simulink model "line_follower_ir"  (R2024b)
settings: Solver=FixedStepDiscrete  StartTime=0.0  StopTime=inf  FixedStep=0.001  RelTol=1e-3  EnableMultiTasking=on
libraries: arduinolib x2
settings Model: ExtModeTrigDuration=2  Creator=$V8IK00-KEIKKPI1645J  LastModifiedBy=$V8IK00-KEIKKPI1645J
settings SolverCC: AutoInsertRateTranBlk=on
settings OptimizationCC: EnhancedBackFolding=on  PassReuseOutputArgsAs=Individual arguments  ZeroExternalMemoryAtStartup=off  ZeroInternalMemoryAtStartup=off  MaxStackSize=64  OptimizeBlockOrder=speed  DifferentSizesBufferReuse=on  OptimizationCustomize=off  EfficientTunableParamExpr=on
settings DebuggingCC: ParameterTunabilityLossMsg=error
settings HardwareCC: ProdBitPerInt=16  ProdBitPerPointer=16  ProdBitPerSizeT=16  ProdBitPerPtrDiffT=16  ProdLargestAtomicFloat=None  ProdWordSize=8  ProdHWDeviceType=Atmel->AVR
settings SFSimCC: MATLABDynamicMemAlloc=off
settings RTWCC: Description=Embedded Coder  SystemTargetFile=ert.tlc  HardwareBoard=Arduino Uno  TemplateMakefile=ert_default_tmf  Toolchain=Arduino AVR  BuildConfiguration=Faster Runs
settings CodeAppCC: ForceParamTrailComments=on  IgnoreCustomStorageClasses=off  OperatorAnnotations=on  SimulinkDataObjDesc=on  SFDataObjDesc=on  InsertBlockDesc=on
settings ERTTargetCC: SupportContinuousTime=on  SupportVariableSizeSignals=on  ExtModeTransport=3  ExtModeStaticAlloc=on  ExtModeAutomaticAllocSize=off  ExtModeStaticAllocSize=250  ExtModeMexFile=ext_xcp  ExtModeIntrfLevel=Level2 - Open  InlinedParameterPlacement=Hierarchical

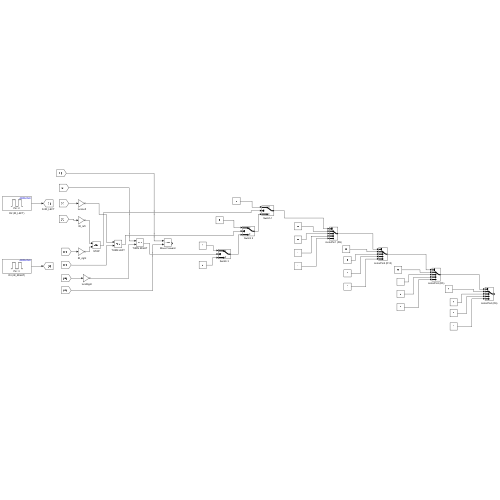
[thumbnail: Simulink's stored preview of the top-level diagram]
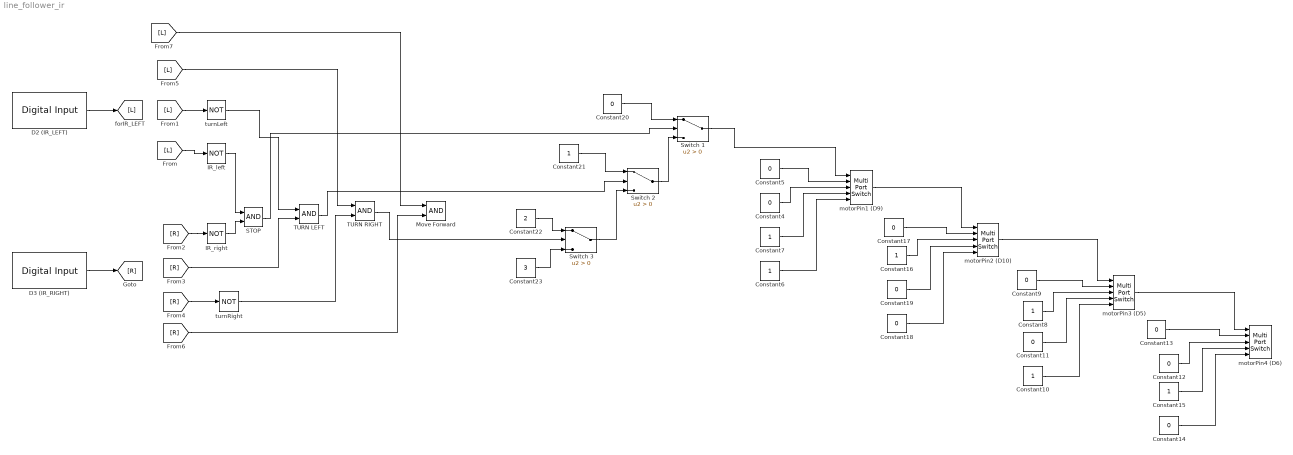
== system line_follower_ir ==
  Constant{6..8,10,15..16,21} (7 alike) : Constant
  Constant{4..5,9,11..14,17..20} (11 alike) : Constant  Value=0
  Constant22 : Constant  Value=2
  Constant23 : Constant  Value=3
  D2 (IR_LEFT) : arduinolib/Digital Input  pinNumber=2  mode=Default  Direction=input  SampleTime=0.1  blockPlatform=arduino
      settings: SourceProductName=Common
  D3 (IR_RIGHT) : arduinolib/Digital Input  pinNumber=3  mode=Default  Direction=input  SampleTime=0.1  blockPlatform=arduino
      settings: SourceProductName=Common
  IR_left : Logic  Operator=NOT  IconShape=distinctive  AllPortsSameDT=off  OutDataTypeStr=boolean
  IR_right : Logic  Operator=NOT  IconShape=distinctive  AllPortsSameDT=off  OutDataTypeStr=boolean
  Move Forward : Logic  AllPortsSameDT=off  OutDataTypeStr=boolean
  STOP : Logic  AllPortsSameDT=off  OutDataTypeStr=boolean
  Switch 1 : Switch  Criteria=u2 > Threshold  SaturateOnIntegerOverflow=off  InputSameDT=off
  Switch 2 : Switch  Criteria=u2 > Threshold  SaturateOnIntegerOverflow=off  InputSameDT=off
  Switch 3 : Switch  Criteria=u2 > Threshold  SaturateOnIntegerOverflow=off  InputSameDT=off
  TURN LEFT : Logic  AllPortsSameDT=off  OutDataTypeStr=boolean
  TURN RIGHT : Logic  AllPortsSameDT=off  OutDataTypeStr=boolean
  motorPin1 (D9) : MultiPortSwitch  DataPortOrder=Zero-based contiguous  Inputs=4  zeroidx=on  SaturateOnIntegerOverflow=off  InputSameDT=off
  motorPin2 (D10) : MultiPortSwitch  DataPortOrder=Zero-based contiguous  Inputs=4  zeroidx=on  SaturateOnIntegerOverflow=off  InputSameDT=off
  motorPin3 (D5) : MultiPortSwitch  DataPortOrder=Zero-based contiguous  Inputs=4  zeroidx=on  SaturateOnIntegerOverflow=off  InputSameDT=off
  motorPin4 (D6) : MultiPortSwitch  DataPortOrder=Zero-based contiguous  Inputs=4  zeroidx=on  SaturateOnIntegerOverflow=off  InputSameDT=off
  turnLeft : Logic  Operator=NOT  IconShape=distinctive  AllPortsSameDT=off  OutDataTypeStr=boolean
  turnRight : Logic  Operator=NOT  IconShape=distinctive  AllPortsSameDT=off  OutDataTypeStr=boolean
  wires:
  D2 (IR_LEFT)/1 -> [L]
  D3 (IR_RIGHT)/1 -> [R]
  IR_right/1 -> STOP/2
  IR_left/1 -> STOP/1
  [L] -> IR_left/1
  [L] -> turnLeft/1
  [R] -> IR_right/1
  [R] -> TURN LEFT/2
  turnLeft/1 -> TURN LEFT/1
  [R] -> turnRight/1
  [L] -> TURN RIGHT/1
  turnRight/1 -> TURN RIGHT/2
  [R] -> Move Forward/2
  [L] -> Move Forward/1
  Constant5/1 -> motorPin1 (D9)/2
  Constant4/1 -> motorPin1 (D9)/3
  Constant7/1 -> motorPin1 (D9)/4
  Constant6/1 -> motorPin1 (D9)/5
  Constant11/1 -> motorPin3 (D5)/4
  Constant8/1 -> motorPin3 (D5)/3
  Constant10/1 -> motorPin3 (D5)/5
  Constant9/1 -> motorPin3 (D5)/2
  Constant15/1 -> motorPin4 (D6)/4
  Constant12/1 -> motorPin4 (D6)/3
  Constant14/1 -> motorPin4 (D6)/5
  Constant13/1 -> motorPin4 (D6)/2
  Constant19/1 -> motorPin2 (D10)/4
  Constant16/1 -> motorPin2 (D10)/3
  Constant18/1 -> motorPin2 (D10)/5
  Constant17/1 -> motorPin2 (D10)/2
  Constant20/1 -> Switch 1/1
  STOP/1 -> Switch 1/2
  Switch 2/1 -> Switch 1/3
  Constant21/1 -> Switch 2/1
  TURN LEFT/1 -> Switch 2/2
  Switch 3/1 -> Switch 2/3
  Constant22/1 -> Switch 3/1
  Constant23/1 -> Switch 3/3
  TURN RIGHT/1 -> Switch 3/2
  Switch 1/1 -> motorPin1 (D9)/1
  motorPin1 (D9)/1 -> motorPin2 (D10)/1
  motorPin2 (D10)/1 -> motorPin3 (D5)/1
  motorPin3 (D5)/1 -> motorPin4 (D6)/1
